simulink model "boost_avg"  (R2026a)
settings: Solver=ode4  StopTime=0.06  FixedStep=1e-07
undefined symbols (not defined in the file): DiscIntNeverNeededParam
settings Model: Creator=matlab-agent-skills  LastModifiedBy=matlab-agent-skills

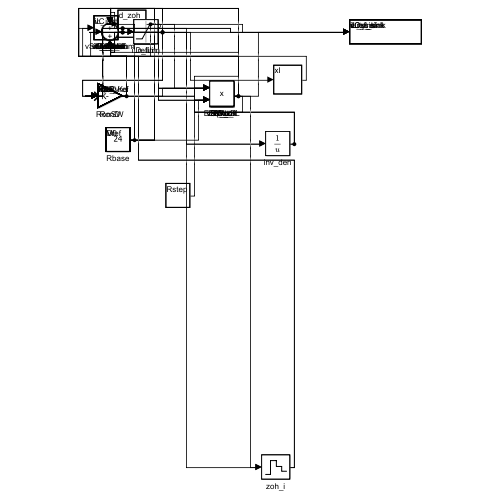
[thumbnail: Simulink's stored preview of the top-level diagram]
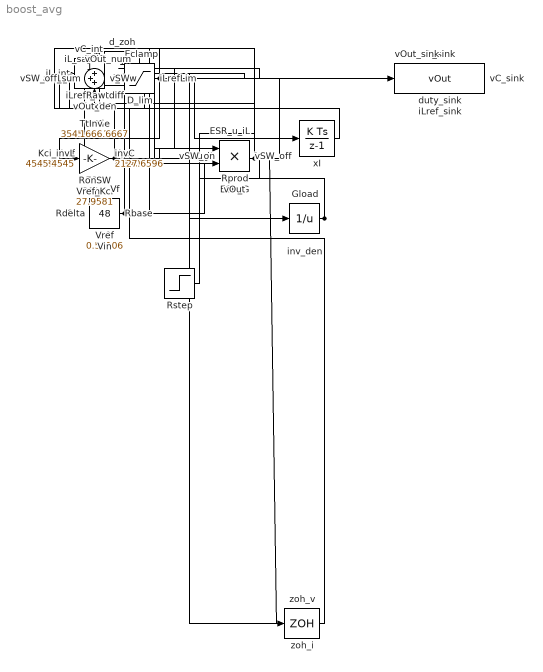
== system boost_avg ==
  D0 : Constant  Value=0.51106
  D_lim : Saturate  UpperLimit=0.9  LowerLimit=0.05
  ESR : Gain  Gain=0.02
  ESR_G : Product
  ESR_u_iL : Product
  Eclamp : Saturate  UpperLimit=2  LowerLimit=-2
  Err : Sum  Inputs=+-
  Gload : Math  Operator=reciprocal
  Kci_Vref : Gain  Gain=0.035768
  Kie : Gain  Gain=3545.6742
  Kpe : Gain  Gain=4.3409
  One : Constant
  RL : Gain  Gain=0.05
  Rbase : Constant  Value=24
  Rdelta : Constant  Value=-8
  Rnow : Sum
  RonD : Gain  Gain=0.02
  RonSW : Gain  Gain=0.02
  Rprod : Product
  Rstep : Step  Time=0.02  SampleTime=0
  TtInv : Gain  Gain=1666.6667
  Vf : Constant  Value=0.5
  Vin : Constant  Value=24
  Vref : Constant  Value=48
  Vref_Kci : Gain  Gain=27.9581
  aw_sum : Sum
  d_raw : Sum
  d_satdiff : Sum  Inputs=+-
  d_zoh : UnitDelay  InitialCondition=0.51106  SampleTime=2e-05
  duty_sink : ToWorkspace  VariableName=duty  SaveFormat=Timeseries  SampleTime=-1
  dxI : Sum
  iC : Sum  Inputs=+-
  iL_err : Sum  Inputs=+-
  iL_int : Integrator  InitialCondition=4.0905
  iL_satdiff : Sum  Inputs=+-
  iL_sink : ToWorkspace  VariableName=iL  SaveFormat=Timeseries  SampleTime=-1
  iLrefLim : Saturate  UpperLimit=8  LowerLimit=0
  iLrefRaw : Sum
  iLref_sink : ToWorkspace  VariableName=iLref  SaveFormat=Timeseries  SampleTime=-1
  iOut : Product
  invC : Gain  Gain=2127.6596
  invL : Gain  Gain=4545.4545
  inv_den : Math  Operator=reciprocal
  u : Sum  Inputs=+-
  u_iL : Product
  vC_int : Integrator  InitialCondition=48
  vC_sink : ToWorkspace  VariableName=vC  SaveFormat=Timeseries  SampleTime=-1
  vL : Sum  Inputs=+--
  vOut : Product
  vOut_den : Sum
  vOut_num : Sum
  vOut_sink : ToWorkspace  VariableName=vOut  SaveFormat=Timeseries  SampleTime=-1
  vSW : Sum
  vSW_off : Product
  vSW_off_sum : Sum  Inputs=+++
  vSW_on : Product
  xI : DiscreteIntegrator  SampleTime=2e-05  ICPrevOutput=DiscIntNeverNeededParam  ICPrevScaledInput=DiscIntNeverNeededParam
  zoh_i : ZeroOrderHold  SampleTime=2e-05
  zoh_v : ZeroOrderHold  SampleTime=2e-05
  wires:
  Rstep/1 -> Rprod/1
  Rdelta/1 -> Rprod/2
  Rbase/1 -> Rnow/1
  Rprod/1 -> Rnow/2
  Rnow/1 -> Gload/1
  One/1 -> u/1, vOut_den/1
  d_zoh/1 -> u/2, vSW_on/1, duty_sink/1
  u/1 -> u_iL/1, vSW_off/1
  iL_int/1 -> u_iL/2, RonSW/1, RonD/1, RL/1, zoh_i/1, iL_sink/1
  ESR/1 -> ESR_u_iL/1, ESR_G/1
  u_iL/1 -> ESR_u_iL/2, iC/1
  vC_int/1 -> vOut_num/1, vC_sink/1
  ESR_u_iL/1 -> vOut_num/2
  Gload/1 -> ESR_G/2, iOut/2
  ESR_G/1 -> vOut_den/2
  vOut_den/1 -> inv_den/1
  vOut_num/1 -> vOut/1
  inv_den/1 -> vOut/2
  vOut/1 -> iOut/1, vSW_off_sum/1, zoh_v/1, vOut_sink/1
  RonSW/1 -> vSW_on/2
  Vf/1 -> vSW_off_sum/2
  RonD/1 -> vSW_off_sum/3
  vSW_off_sum/1 -> vSW_off/2
  vSW_on/1 -> vSW/1
  vSW_off/1 -> vSW/2
  Vin/1 -> vL/1
  vSW/1 -> vL/2
  RL/1 -> vL/3
  vL/1 -> invL/1
  invL/1 -> iL_int/1
  iOut/1 -> iC/2
  iC/1 -> invC/1
  invC/1 -> vC_int/1
  Vref/1 -> Err/1
  zoh_v/1 -> Err/2
  Err/1 -> Eclamp/1
  Eclamp/1 -> Kpe/1, Kie/1
  Kpe/1 -> iLrefRaw/1
  iLrefRaw/1 -> iLrefLim/1, iL_satdiff/2
  iLrefLim/1 -> iL_satdiff/1, iL_err/1, iLref_sink/1
  zoh_i/1 -> iL_err/2
  iL_err/1 -> Kci_Vref/1
  Kci_Vref/1 -> d_raw/1
  D0/1 -> d_raw/2
  d_raw/1 -> D_lim/1, d_satdiff/2
  D_lim/1 -> d_zoh/1, d_satdiff/1
  d_satdiff/1 -> Vref_Kci/1
  Vref_Kci/1 -> aw_sum/1
  iL_satdiff/1 -> aw_sum/2
  aw_sum/1 -> TtInv/1
  Kie/1 -> dxI/1
  TtInv/1 -> dxI/2
  dxI/1 -> xI/1
  xI/1 -> iLrefRaw/2
